simulink model "System_D_simulink"  (R2026a)
settings: Solver=ode23t  StopTime=0.45  MaxStep=1/(2*fs)  RelTol=1e-5
model workspace (MAT data in the model file):
  Cmid = 6.8e-06
  Ctw = 5.6e-06
  Lmid = 0.00082
  Ltw = 0.00022
  Rp = 3.3
  Rs = 4.7
  a_hp = [1 -1.96992019814 0.970365941122]
  a_lp = [1 -1.96992019814 0.970365941122]
  b_hp = [0.985071534816 -1.97014306963 0.985071534816]
  b_lp = [0.000111435745339 0.000222871490678 0.000111435745339]
  delay_samples = 16384
  f = [50; 51; 52; 53; 54; 55; 56; 57; 58; 59; 60; 61; 62; 63; 64; 65; 66; 67; 68; 69; 70; 71; 72; 73; 74; 75; 77; 78; 79; 80; 81; 82; 83; 85; 86; 87; 88; 90; 91; 92; 94; 95; 96; 98; 99; 101; 102; 104; 105; 107; 108; 110; 111; 113; 115; 116; 118; 120; 121; 123; 125; 127; 129; 131; 132; 134; 136; 138; 140; 142; 144; 147; 149; 151; 153; 155; 157; 160; 162; 164; 167; 169; 172; 174; 177; 179; 182; 185; 187; 190; 193; 196; 198; 201; 204; 207; 210; 213; 216; 220; 223; 226; 229; 233; 236; 239; 243; 246; 250; 254; 257; 261; 265; 269; 273; 277; 281; 285; 289; 293; 297; 302; 306; 310; 315; 320; 324; 329; 334; 339; 343; 348; 354; 359; 364; 369; 375; 380; 386; 391; 397; 403; 408; 414; 420; 427; 433; 439; 445; 452; 459; 465; 472; 479; 486; 493; 500; 507; 515; 522; 530; 537; 545; 553; 561; 569; 578; 586; 595; 603; 612; 621; 630; 639; 648; 658; 667; 677; 687; 697; 707; 717; 728; 738; 749; 760; 771; 782; 794; 805; 817; 829; 841; 853; 866; 878; 891; 904; 917; 930; 944; 958; 972; 986; 1000; 1015; 1029; 1044; 1059; 1075; 1090; 1106; 1122; 1138; 1155; 1172; 1189; 1206; 1223; 1241; 1259; 1277; 1296; 1315; 1334; 1353; 1373; 1393; 1413; 1433; 1454; 1475; 1497; 1518; 1540; 1563; 1585; 1608; 1632; 1655; 1679; 1704; 1729; 1754; 1779; 1805; 1831; 1858; 1885; 1912; 1940; 1968; 1996; 2025; 2055; 2085; 2115; 2145; 2177; 2208; 2240; 2273; 2306; 2339; 2373; 2407; 2442; 2478; 2514; 2550; 2587; 2625; 2663; 2701; 2741; 2780; 2821; 2862; 2903; 2945; 2988; 3031; 3075; 3120; 3165; 3211; 3258; 3305; 3353; 3402; 3451; 3501; 3552; 3603; 3655; 3709; 3762; 3817; 3872; 3928; 3985; 4043; 4102; 4161; 4222; 4283; 4345; 4408; 4472; 4537; 4603; 4670; 4737; 4806; 4876; 4947; 5018; 5091; 5165; 5240; 5316; 5393; 5471; 5551; 5631; 5713; 5796; 5880; 5965; 6052; 6139; 6228; 6319; 6410; 6503; 6598; 6694; 6791; 6889; 6989; 7090; 7193; 7298; 7404; 7511; 7620; 7730; 7843; 7956; 8072; 8189; 8308; 8428; 8550; 8674; 8800; 8928; 9057; 9189; 9322; 9457; 9595; 9734; 9875; 10018; 10164; 10311; 10461; 10612; 10766; 10922; 11081; 11242; 11405; 11570; 11738; 11908; 12081; 12256; 12434; 12615; 12798; 12983; 13172; 13363; 13556; 13753; 13953; 14155; 14360; 14569; 14780; 14994; 15212; 15433; 15657; 15884; 16114; 16348; 16585; 16826; 17070; 17317; 17569; 17823; 18082; 18344; 18610; 18880; 19154; 19432; 19714]
  fir_mid = [2.88615785051e-06 2.87905807458e-06 2.86601289236e-06 2.86209989692e-06 2.87914488669e-06 2.90760278468e-06 2.91495292008e-06 2.86191467289e-06 2.72461541069e-06 2.51079055348e-06 2.26185413326e-06 2.03723101733e-06 ... (32768 elements, 1x32768)]
  fir_tw = [-2.60624232609e-06 -2.27215528381e-06 -2.25731305883e-06 -2.5961984087e-06 -2.98688820194e-06 -3.09958236215e-06 -2.8639414963e-06 -2.40425500843e-06 -1.83630123021e-06 -1.24253482671e-06 -7.49249289368e-07 -4.94473143896e-07 ... (32768 elements, 1x32768)]
  fir_woof = [2.71744577313e-06 2.91995199079e-06 3.2994659548e-06 3.73731262893e-06 4.11733049488e-06 4.36319861388e-06 4.44606576447e-06 4.38093146601e-06 4.22485207588e-06 4.06866670403e-06 4.00752757287e-06 4.09493136226e-06 ... (32768 elements, 1x32768)]
  fs = 96000
  g_woof = 0.595662143529
  pol_mid = 1
  pol_tw = 1
  pol_woof = 1
  ref_mid_im = [-2.02471473106e-05 -2.97451137892e-05 -8.18998441469e-06 -9.44112206059e-06 -9.98474521822e-06 -1.80323069699e-05 -2.36335585807e-05 -2.07669965717e-05 -2.44493768902e-05 1.53522925063e-05 1.26835054665e-05 -2.72017381443e-05 ... (412 elements, 412x1)]
  ref_mid_re = [5.11138743346e-05 5.27646175102e-05 6.43853406534e-05 7.19878043236e-05 9.07552490467e-05 9.02364974629e-05 0.000108111340774 0.000127641838401 0.000164076149146 0.00016525070791 0.000233272470596 0.000266015581949 ... (412 elements, 412x1)]
  ref_sum_im = [-0.237822623935 -0.249208923528 -0.252704050496 -0.277443609145 -0.287425433384 -0.281925307353 -0.273684166346 -0.301968651196 -0.32702532988 -0.356393021871 -0.384013551582 -0.427201303434 ... (412 elements, 412x1)]
  ref_sum_re = [0.0079461204201 -0.00807298700672 0.0366054479648 0.0304994442536 0.00185490294456 0.00396661293164 0.0289494720887 0.0412739478932 0.0471470600314 0.0668622907578 0.0743628077169 0.0739295887598 ... (412 elements, 412x1)]
  ref_tw_im = [2.66562025616e-10 1.06047214067e-10 3.29547259586e-10 9.1080418365e-11 1.01471933591e-10 -1.2721995912e-10 -3.07463357353e-10 -9.90286820009e-10 -4.40391607082e-10 -7.61622541983e-10 -4.0356932662e-10 2.86227803489e-10 ... (412 elements, 412x1)]
  ref_tw_re = [-2.81565378421e-10 4.5611348125e-11 -1.70188531961e-10 -5.4214307034e-11 1.59527809471e-12 1.81051243455e-11 4.85092069489e-10 1.65769684723e-11 -4.00879085044e-10 1.05530110859e-10 -9.04825296789e-10 -1.29396251722e-09 ... (412 elements, 412x1)]
  ref_woof_im = [-0.237802377054 -0.24917917852 -0.252695860841 -0.277434168114 -0.28741544874 -0.281907274919 -0.27366053248 -0.301947883209 -0.327000880063 -0.356408373402 -0.384026234684 -0.427174101982 ... (412 elements, 412x1)]
  ref_woof_re = [0.00789500682733 -0.00812575166984 0.0365410627943 0.0304274565035 0.00176414769392 0.00387637641607 0.0288413602628 0.0411463060382 0.0469829842831 0.0666970399443 0.0741295361511 0.0736635744718 ... (412 elements, 412x1)]
  tf_mid = [0.0998356483895+0.00966008754272i 0.102076870231-0.00313844645705i 0.0946421894936+0.0361663561834i 0.0979510358274+0.0379690093634i 0.112990905181+0.0477044018154i 0.109044667147+0.03621348334i 0.122419200152+0.0393998382701i 0.130377482303+0.0511658321292i 0.15467322795+0.064682478583i 0.125179778541+0.0942375054511i 0.168395608846+0.119101574545i 0.197284206678+0.0996824269753i ... (412 elements, 412x1)]
  tf_mid_im = [0.00966008754272 -0.00313844645705 0.0361663561834 0.0379690093634 0.0477044018154 0.03621348334 0.0393998382701 0.0511658321292 0.064682478583 0.0942375054511 0.119101574545 0.0996824269753 ... (412 elements, 412x1)]
  tf_mid_re = [0.0998356483895 0.102076870231 0.0946421894936 0.0979510358274 0.112990905181 0.109044667147 0.122419200152 0.130377482303 0.15467322795 0.125179778541 0.168395608846 0.197284206678 ... (412 elements, 412x1)]
  tf_tw = [0.0198457022563-0.00715469241983i 8.34206280492e-05-0.00557696831399i 0.012563148971-0.00982739097113i 0.00336856881883-0.00227734746733i 0.00145980497416-0.00315933910186i -0.00222599627599+0.00326018180298i -0.0157604599169+0.00155018479379i -0.0116189930625+0.0216379610708i 0.00333344091506+0.0128808016901i -0.00916110563484+0.0125093739866i 0.0108979357018+0.0144059793721i 0.0209366637571+0.00636489608235i ... (412 elements, 412x1)]
  tf_tw_im = [-0.00715469241983 -0.00557696831399 -0.00982739097113 -0.00227734746733 -0.00315933910186 0.00326018180298 0.00155018479379 0.0216379610708 0.0128808016901 0.0125093739866 0.0144059793721 0.00636489608235 ... (412 elements, 412x1)]
  tf_tw_re = [0.0198457022563 8.34206280492e-05 0.012563148971 0.00336856881883 0.00145980497416 -0.00222599627599 -0.0157604599169 -0.0116189930625 0.00333344091506 -0.00916110563484 0.0108979357018 0.0209366637571 ... (412 elements, 412x1)]
  tf_woof = [0.181608417788-0.356022917871i 0.168786108916-0.383280529798i 0.242166050712-0.354017107262i 0.254795120302-0.393610885978i 0.223128594979-0.428249167557i 0.225804856879-0.416417838149i 0.259960687795-0.382374342555i 0.304360000511-0.411814390306i 0.337174588175-0.441052500026i 0.394426682217-0.464522244478i 0.432789825657-0.494799805707i 0.473682687703-0.553647303077i ... (412 elements, 412x1)]
  tf_woof_im = [-0.356022917871 -0.383280529798 -0.354017107262 -0.393610885978 -0.428249167557 -0.416417838149 -0.382374342555 -0.411814390306 -0.441052500026 -0.464522244478 -0.494799805707 -0.553647303077 ... (412 elements, 412x1)]
  tf_woof_re = [0.181608417788 0.168786108916 0.242166050712 0.254795120302 0.223128594979 0.225804856879 0.259960687795 0.304360000511 0.337174588175 0.394426682217 0.432789825657 0.473682687703 ... (412 elements, 412x1)]
  zi_mid_im = [3.15145569017 3.226811686 3.32611598161 3.44333048105 3.54533776416 3.64854828115 3.76283446092 3.89289495957 4.01551140677 4.150592994 4.29260801654 4.46368784868 ... (412 elements, 412x1)]
  zi_mid_re = [5.31943483026 5.378404173 5.39638717148 5.47983267484 5.52299089563 5.59239183084 5.67547146448 5.74779130072 5.80510938691 5.884400566 5.98099909956 6.07160964327 ... (412 elements, 412x1)]
  zi_tw_im = [0.3929867032 0.3929867032 0.3929867032 0.3929867032 0.3929867032 0.3929867032 0.3929867032 0.3929867032 0.3929867032 0.3929867032 0.3929867032 0.3929867032 ... (412 elements, 412x1)]
  zi_tw_re = [3.639639303 3.639639303 3.639639303 3.639639303 3.639639303 3.639639303 3.639639303 3.639639303 3.639639303 3.639639303 3.639639303 3.639639303 ... (412 elements, 412x1)]
libraries: fl_lib x25, nesl_utility x5
(part 1 of 2)
settings Model: Creator=mads  LastModifiedBy=mads

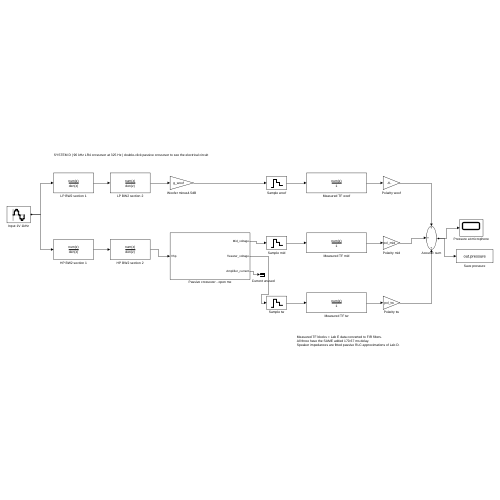
[thumbnail: Simulink's stored preview of the top-level diagram]
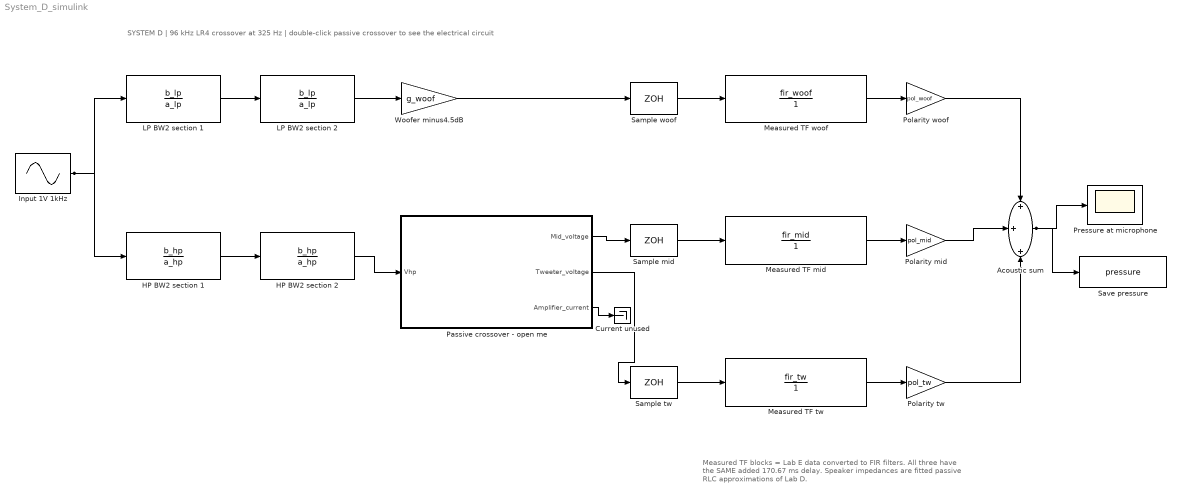
== system System_D_simulink ==
  note: SYSTEM D | 96 kHz LR4 crossover at 325 Hz | double-click passive crossover to see the electrical circuit
  note: Measured TF blocks = Lab E data converted to FIR filters.
      | All three have the SAME added 170.67 ms delay.
      | Speaker impedances are fitted passive RLC approximations of Lab D.
  Acoustic sum : Sum  Inputs=+++
  Current unused : Terminator
  HP BW2 section 1 : DiscreteFilter  Numerator=b_hp  Denominator=a_hp  SampleTime=1/fs
  HP BW2 section 2 : DiscreteFilter  Numerator=b_hp  Denominator=a_hp  SampleTime=1/fs
  Input 1V 1kHz : Sin  Frequency=2*pi*1000  SampleTime=1/fs
  LP BW2 section 1 : DiscreteFilter  Numerator=b_lp  Denominator=a_lp  SampleTime=1/fs
  LP BW2 section 2 : DiscreteFilter  Numerator=b_lp  Denominator=a_lp  SampleTime=1/fs
  Measured TF mid : DiscreteFilter  Numerator=fir_mid  Denominator=1  SampleTime=1/fs
  Measured TF tw : DiscreteFilter  Numerator=fir_tw  Denominator=1  SampleTime=1/fs
  Measured TF woof : DiscreteFilter  Numerator=fir_woof  Denominator=1  SampleTime=1/fs
  Passive crossover - open me : Subsystem
  Polarity mid : Gain  Gain=pol_mid
  Polarity tw : Gain  Gain=pol_tw
  Polarity woof : Gain  Gain=pol_woof
  Pressure at microphone : Scope
  Sample mid : ZeroOrderHold  SampleTime=1/fs
  Sample tw : ZeroOrderHold  SampleTime=1/fs
  Sample woof : ZeroOrderHold  SampleTime=1/fs
  Save pressure : ToWorkspace  VariableName=pressure  SaveFormat=Timeseries  SampleTime=-1
  Woofer minus4.5dB : Gain  Gain=g_woof
  wires:
  Input 1V 1kHz/1 -> LP BW2 section 1/1, HP BW2 section 1/1
  LP BW2 section 1/1 -> LP BW2 section 2/1
  HP BW2 section 1/1 -> HP BW2 section 2/1
  LP BW2 section 2/1 -> Woofer minus4.5dB/1
  HP BW2 section 2/1 -> Passive crossover - open me/1(Vhp)
  Passive crossover - open me/3(Amplifier_current) -> Current unused/1
  Sample woof/1 -> Measured TF woof/1
  Measured TF woof/1 -> Polarity woof/1
  Sample mid/1 -> Measured TF mid/1
  Measured TF mid/1 -> Polarity mid/1
  Sample tw/1 -> Measured TF tw/1
  Measured TF tw/1 -> Polarity tw/1
  Woofer minus4.5dB/1 -> Sample woof/1
  Passive crossover - open me/1(Mid_voltage) -> Sample mid/1
  Passive crossover - open me/2(Tweeter_voltage) -> Sample tw/1
  Polarity woof/1 -> Acoustic sum/1
  Polarity mid/1 -> Acoustic sum/2
  Polarity tw/1 -> Acoustic sum/3
  Acoustic sum/1 -> Pressure at microphone/1, Save pressure/1
